simulink model "buck_ADRC_MBD_NPU_24b"  (R2025b)
settings: Solver=FixedStepAuto  StartTime=0.0  StopTime=Inf  RelTol=1e-3  EnableMultiTasking=on
InitFcn:
  | run(fullfile(fileparts(get_param(bdroot,'FileName')),'buck_npu_load_workspace.m'));
model workspace (MAT data in the model file):
  II = 0.000447333333333
  IP = 0.02847
undefined symbols (not defined in the file or in its folder): bit, Down, GPTRIP1SEL, TZ1, Up
libraries: c2802xlib x10, slpidlib x4, c28P55xlib x3, c2000lib x1
Description:
  | H15 full-convolution NPU integration: continuous 30 kHz history; background normalization/launch/result scheduling; matched-target-only LADRC correction. Boot: alpha=0, enable=1, NPU run disabled.
settings Model: ExtModeTrigDuration=8  Creator=User  LastModifiedBy=34109
settings OptimizationCC: DefaultParameterBehavior=Inlined  DefaultUnderspecifiedDataType=single  EnhancedBackFolding=on  PassReuseOutputArgsAs=Individual arguments  MaxStackSize=1024  OptimizeBlockOrder=speed  DifferentSizesBufferReuse=on  OptimizationCustomize=off  EfficientTunableParamExpr=on
settings DebuggingCC: ParameterTunabilityLossMsg=error
settings HardwareCC: ProdBitPerChar=16.0  ProdBitPerInt=16.0  ProdBitPerPointer=32.0  ProdBitPerSizeT=32.0  ProdBitPerPtrDiffT=32.0  ProdLargestAtomicInteger=Integer  ProdLargestAtomicFloat=None  ProdWordSize=16.0  ProdLongLongMode=on  ProdHWDeviceType=Texas Instruments->C2000  HardwareBoardFeatureSet=SoCBlockset
settings SFSimCC: MATLABDynamicMemAlloc=off
settings RTWCC: SystemTargetFile=ert.tlc  HardwareBoard=TI F28P55x  TemplateMakefile=ert_default_tmf  PostCodeGenCommand=buck_npu_post_codegen(buildInfo); codertarget.postCodeGenHookCommand(h);  CustomInitializer=buck_npu_platform_init();  Toolchain=Texas Instruments Code Composer Studio - EABI (C2000)  CodeProfilingSaveOptions=MetricsOnly  Description=Embedded Coder
settings RTWCC: CustomHeaderCode=|
  | #include "buck_npu.h"
  | #include "buck_npu_platform.h"
settings RTWCC: CustomInclude=|
  | C:\Users\34109\Desktop\delivery_file\F28P55_v16
  | D:/ti/c2000/C2000Ware_26_02_00_00/device_support/f28p55x/common/include
  | D:/ti/c2000/C2000Ware_26_02_00_00/driverlib/f28p55x/driverlib
settings RTWCC: CustomSource=|
  | C:\Users\34109\Desktop\delivery_file\F28P55_v16\buck_npu.c
  | C:\Users\34109\Desktop\delivery_file\F28P55_v16\buck_npu_sdk_port.c
  | C:\Users\34109\Desktop\delivery_file\F28P55_v16\buck_npu_platform.c
  | C:\Users\34109\Desktop\delivery_file\F28P55_v16\buck_load_observer.c
  | C:\Users\34109\Desktop\delivery_file\F28P55_v16\buck_npu_compensation.c
settings RTWCC: CustomLibrary=|
  | C:\Users\34109\Desktop\delivery_file\F28P55_v16\mod.a
  | C:\Users\34109\Desktop\delivery_file\F28P55_v16\buck_npu_sections.cmd
settings CodeAppCC: ForceParamTrailComments=on  IgnoreCustomStorageClasses=off  OperatorAnnotations=on  SimulinkDataObjDesc=on  SFDataObjDesc=on  InsertBlockDesc=on
settings ERTTargetCC: ExtModeTransport=4.0  ExtModeStaticAlloc=on  ExtModeAutomaticAllocSize=off  ExtModeStaticAllocSize=10000.0  ExtModeMexFile=ext_xcp  ExtModeIntrfLevel=Level2 - Open  EnableUserReplacementTypes=on  CodeReplacementLibrary=TI C28x

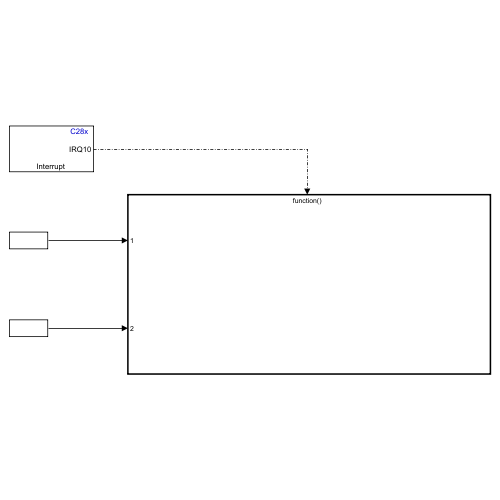
[thumbnail: Simulink's stored preview of the top-level diagram]
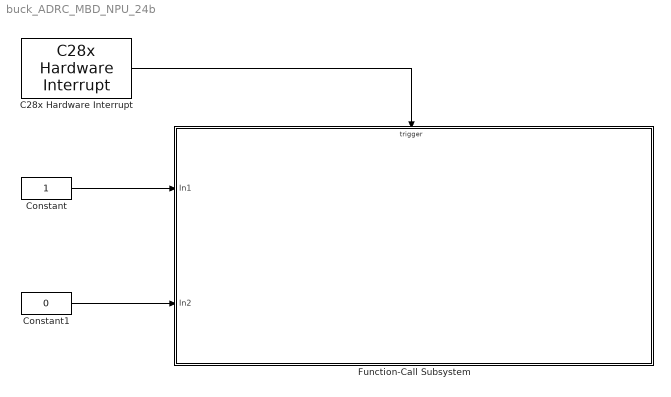
== system buck_ADRC_MBD_NPU_24b ==
  C28x Hardware Interrupt : c2000lib/Scheduling/C28x Hardware Interrupt  irqnumbers=[10]  pienumbers=[4]  irqpriorities=[30]  irqpreempts=[0]  showinput=off  dspchiptype=C280X
  Constant : Constant
  Constant1 : Constant  Value=0
  Function-Call Subsystem : Subsystem  TreatAsAtomicUnit=on
  wires:
  C28x Hardware Interrupt/1 -> Function-Call Subsystem/Trigger
  Constant1/1 -> Function-Call Subsystem/2(In2)
  Constant/1 -> Function-Call Subsystem/1(In1)

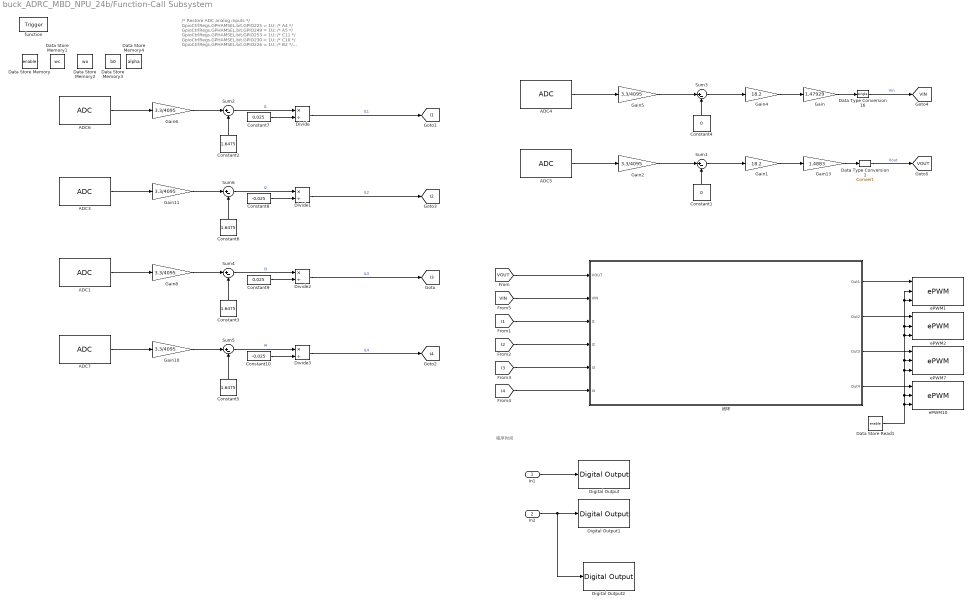
== system buck_ADRC_MBD_NPU_24b/Function-Call Subsystem ==
  note: /* Restore ADC analog inputs */
      |   GpioCtrlRegs.GPHAMSEL.bit.GPIO225 = 1U;  /* A4  */
      |   GpioCtrlRegs.GPHAMSEL.bit.GPIO249 = 1U;  /* A5  */
      |   GpioCtrlRegs.GPHAMSEL.bit.GPIO253 = 1U;  /* C11 */
      |   GpioCtrlRegs.GPHAMSEL.bit.GPIO230 = 1U;  /* C10 */
      |   GpioCtrlRegs.GPHAMSEL.bit.GPIO226 = 1U;  /* B2  */
      |   GpioCtrlRegs.GPHAMSEL.bit.GPIO237 = 1U;  /* B10 */
  note: 程序时间
  In1 : Inport
  In2 : Inport  Port=2
  function : TriggerPort  TriggerType=function-call  VariantControl=(inherit)
  ADC1 : c2802xlib/ADC  blkParamProc=C2000_Type6  ADCModule=A  samplingMode=Single sample mode  ADCResolution=12-bit (Single-ended input)  ADC29xResolution=12-bit  ADCMode=Single-ended input  useSOC1=SOC0  useSOC2=SOC0_SOC1  SOCAcquisitionWindow=56  SOCTriggerSource=ePWM7_ADCSOCA  SOCInterruptTrigger=No ADCINT  Ts=-1  dType=single  postInterrupt=off  interruptSel=ADCINT1  ADCINTContinuous=off  endma=off  chdma=1  conv1=ADCINA0  conv2=ADCINA0 and ADCINB0  conv1_Type4=ADCIN5  conv2_Type4=ADCIN0 and ADCIN1
      settings: LibrarySourceBlock=c28P55xlib/ADC
  ADC3 : c2802xlib/ADC  blkParamProc=C2000_Type6  ADCModule=C  samplingMode=Single sample mode  ADCResolution=12-bit (Single-ended input)  ADC29xResolution=12-bit  ADCMode=Single-ended input  useSOC1=SOC1  useSOC2=SOC0_SOC1  SOCAcquisitionWindow=56  SOCTriggerSource=ePWM2_ADCSOCA  SOCInterruptTrigger=No ADCINT  Ts=-1  dType=single  postInterrupt=off  interruptSel=ADCINT1  ADCINTContinuous=off  endma=off  chdma=1  conv1=ADCINA0  conv2=ADCINA0 and ADCINB0  conv1_Type4=ADCIN10  conv2_Type4=ADCIN0 and ADCIN1
      settings: LibrarySourceBlock=c28P55xlib/ADC
  ADC4 : c2802xlib/ADC  blkParamProc=C2000_Type6  ADCModule=B  samplingMode=Single sample mode  ADCResolution=12-bit (Single-ended input)  ADC29xResolution=12-bit  ADCMode=Single-ended input  useSOC1=SOC0  useSOC2=SOC0_SOC1  SOCAcquisitionWindow=56  SOCTriggerSource=ePWM1_ADCSOCA  SOCInterruptTrigger=No ADCINT  Ts=-1  dType=single  postInterrupt=off  interruptSel=ADCINT1  ADCINTContinuous=off  endma=off  chdma=1  conv1=ADCINA0  conv2=ADCINA0 and ADCINB0  conv1_Type4=ADCIN2  conv2_Type4=ADCIN0 and ADCIN1
      settings: LibrarySourceBlock=c28P55xlib/ADC
  ADC5 : c2802xlib/ADC  blkParamProc=C2000_Type6  ADCModule=B  samplingMode=Single sample mode  ADCResolution=12-bit (Single-ended input)  ADC29xResolution=12-bit  ADCMode=Single-ended input  useSOC1=SOC1  useSOC2=SOC0_SOC1  SOCAcquisitionWindow=56  SOCTriggerSource=ePWM1_ADCSOCA  SOCInterruptTrigger=No ADCINT  Ts=-1  dType=single  postInterrupt=off  interruptSel=ADCINT1  ADCINTContinuous=on  endma=off  chdma=1  conv1=ADCINA0  conv2=ADCINA0 and ADCINB0  conv1_Type4=ADCIN10  conv2_Type4=ADCIN0 and ADCIN1
      settings: LibrarySourceBlock=c28P55xlib/ADC
  ADC6 : c2802xlib/ADC  blkParamProc=C2000_Type6  ADCModule=C  samplingMode=Single sample mode  ADCResolution=12-bit (Single-ended input)  ADC29xResolution=12-bit  ADCMode=Single-ended input  useSOC1=SOC0  useSOC2=SOC0_SOC1  SOCAcquisitionWindow=56  SOCTriggerSource=ePWM1_ADCSOCA  SOCInterruptTrigger=No ADCINT  Ts=-1  dType=single  postInterrupt=off  interruptSel=ADCINT1  ADCINTContinuous=off  endma=off  chdma=1  conv1=ADCINA0  conv2=ADCINA0 and ADCINB0  conv1_Type4=ADCIN11  conv2_Type4=ADCIN0 and ADCIN1
      settings: LibrarySourceBlock=c28P55xlib/ADC
  ADC7 : c2802xlib/ADC  blkParamProc=C2000_Type6  ADCModule=A  samplingMode=Single sample mode  ADCResolution=12-bit (Single-ended input)  ADC29xResolution=12-bit  ADCMode=Single-ended input  useSOC1=SOC1  useSOC2=SOC0_SOC1  SOCAcquisitionWindow=56  SOCTriggerSource=ePWM10_ADCSOCA  SOCInterruptTrigger=No ADCINT  Ts=-1  dType=single  postInterrupt=on  interruptSel=ADCINT4  ADCINTContinuous=on  endma=off  chdma=1  conv1=ADCINA0  conv2=ADCINA0 and ADCINB0  conv1_Type4=ADCIN4  conv2_Type4=ADCIN0 and ADCIN1
      settings: LibrarySourceBlock=c28P55xlib/ADC
  Constant1 : Constant  Value=0  OutDataTypeStr=single
  Constant10 : Constant  Value=-0.025
  Constant{2..3,5..6} (4 alike) : Constant  Value=1.6475  OutDataTypeStr=single
  Constant4 : Constant  Value=0  OutDataTypeStr=single
  Constant7 : Constant  Value=0.025
  Constant8 : Constant  Value=-0.025
  Constant9 : Constant  Value=0.025
  Data Store Memory : DataStoreMemory  DataStoreName=enable  WriteAfterWriteMsg=warning  InitialValue=1  ShowAdditionalParam=off  StateMustResolveToSignalObject=on
  Data Store Memory1 : DataStoreMemory  DataStoreName=wc  WriteAfterWriteMsg=warning  InitialValue=5000  ShowAdditionalParam=off  StateMustResolveToSignalObject=on
  Data Store Memory2 : DataStoreMemory  DataStoreName=wo  WriteAfterWriteMsg=warning  InitialValue=14000  ShowAdditionalParam=off  StateMustResolveToSignalObject=on
  Data Store Memory3 : DataStoreMemory  DataStoreName=b0  WriteAfterWriteMsg=warning  InitialValue=20000  ShowAdditionalParam=off  StateMustResolveToSignalObject=on
  Data Store Memory4 : DataStoreMemory  DataStoreName=alpha  WriteAfterWriteMsg=warning  ShowAdditionalParam=off  StateMustResolveToSignalObject=on
  Data Store Read1 : DataStoreRead  DataStoreName=enable  IndexOptions=Index vector (dialog)  Indices=1  OutputSizes=1
  Data Type Conversion1 : DataTypeConversion  SaturateOnIntegerOverflow=off  RndMeth=Floor
  Data Type Conversion16 : DataTypeConversion  OutDataTypeStr=single  SaturateOnIntegerOverflow=off  RndMeth=Floor
  Digital Output : c28P55xlib/Digital Output  ExecutionOrder=First  GPIO_Number=GPIO16~GPIO23  GPIO_Bit0=off  GPIO_BIT0_Toggle=off  GPIO_Bit1=off  GPIO_BIT1_Toggle=off  GPIO_Bit2=off  GPIO_BIT2_Toggle=off  GPIO_Bit3=off  GPIO_BIT3_Toggle=off  GPIO_Bit4=off  GPIO_BIT4_Toggle=off  GPIO_Bit5=off  GPIO_BIT5_Toggle=off  GPIO_Bit6=on  GPIO_BIT6_Toggle=off  GPIO_Bit7=off  GPIO_BIT7_Toggle=off
  Digital Output1 : c28P55xlib/Digital Output  ExecutionOrder=Last  GPIO_Number=GPIO16~GPIO23  GPIO_Bit0=off  GPIO_BIT0_Toggle=off  GPIO_Bit1=off  GPIO_BIT1_Toggle=off  GPIO_Bit2=off  GPIO_BIT2_Toggle=off  GPIO_Bit3=off  GPIO_BIT3_Toggle=off  GPIO_Bit4=off  GPIO_BIT4_Toggle=off  GPIO_Bit5=off  GPIO_BIT5_Toggle=off  GPIO_Bit6=on  GPIO_BIT6_Toggle=off  GPIO_Bit7=off  GPIO_BIT7_Toggle=off
  Digital Output2 : c28P55xlib/Digital Output  GPIO_Number=GPIO56~GPIO63  GPIO_Bit0=off  GPIO_BIT0_Toggle=off  GPIO_Bit1=off  GPIO_BIT1_Toggle=off  GPIO_Bit2=off  GPIO_BIT2_Toggle=off  GPIO_Bit3=off  GPIO_BIT3_Toggle=off  GPIO_Bit4=off  GPIO_BIT4_Toggle=off  GPIO_Bit5=off  GPIO_BIT5_Toggle=off  GPIO_Bit6=off  GPIO_BIT6_Toggle=off  GPIO_Bit7=on  GPIO_BIT7_Toggle=off
  Divide{,1..3} (4 alike) : Product  Inputs=*/
  Gain : Gain  Gain=1.47929
  Gain1 : Gain  Gain=18.2
  Gain{2,5..6,8,10..11} (6 alike) : Gain  Gain=3.3/4095
  Gain13 : Gain  Gain=1.4883
  Gain4 : Gain  Gain=18.2
  Sum{1..6} (6 alike) : Sum  Inputs=|+-
  ePWM1 : c2802xlib/ePWM  PwmType=C2000_Type4_F28002x  useModule=ePWM1  ePWMxLINKTBPRD=Not Linked  periodUnits=Clock cycles  timerSource=Specify via dialog  timerPeriod_clk=2500  timerPeriod_sec=0.0001  tbshadow=Counter equals to zero  countingMode=Up-Down  phaseActiveEnable=Disable  phaseDirection=Count down after sync  phaseActive=0  synchronizationEnable=off  dcaevt1Sync=off  dcbevt1Sync=off  synchronizationOption=Disable  dcbevt1SyncOut=off  dcaevt1SyncOut=off  cmpdSyncOut=off  cmpcSyncOut=off  cmpbSyncOut=off  zeroSyncOut=on  swfSyncOut=off  perSynchronizationOption=Counter equals to period (CTR=PRD)  clockPrescale=1  HSclockPrescale=1  enswap=off  ePWMxAStatus=on  ePWMxAactionLogic1=Set  ePWMxAactionLogic2=Do nothing  ePWMxAactionLogic3=Clear  ePWMxAactionLogic4=Set  ePWMxAactionLogic5=Do nothing  ePWMxAactionLogic6=Do nothing  ePWMxACSFenable=on  ePWMxACSFvalue=Forcing disable  ePWMxASFreload=Zero  ePWMxBStatus=off  ePWMxBactionLogic1=Set  ePWMxBactionLogic2=Clear  ePWMxBactionLogic3=Do nothing  ePWMxBactionLogic4=Do nothing  ePWMxBactionLogic5=Clear  ePWMxBactionLogic6=Set  ePWMxBCSFenable=on  ePWMxBCSFvalue=Forcing disable  ePWMxBSFreload=Zero  ePWNxBOutWay=off  ePWMxLINKCMPA=Not Linked  CMPAUnits=Percentages  CMPASource=Input port  CMPAValue_per=50  CMPAValue_clk=2500  enCMPAshadow=Counter equals to zero (CTR=Zero)  ePWMxLINKCMPB=Not Linked  CMPBUnits=Clock cycles  CMPBSource=Specify via dialog  CMPBValue_per=50  CMPBValue_clk=32000  enCMPBshadow=Counter equals to zero (CTR=Zero)  ePWMxLINKCMPC=Not Linked  CMPCUnits=Clock cycles  CMPCSource=Specify via dialog  CMPCValue_per=50  CMPCValue_clk=32000  enCMPCshadow=Counter equals to zero (CTR=Zero)  ePWMxLINKCMPD=Not Linked  CMPDUnits=Clock cycles  CMPDSource=Specify via dialog  CMPDValue_per=50  CMPDValue_clk=32000  enCMPDshadow=Counter equals to zero (CTR=Zero)  enableDBePWMxA=on  enableDBePWMxB=on  enhalfcycle=off  DBpolarity=Active high complementary (AHC)  DBedgeDelay=Positive  DBSource_ePWMxA=ePWMxA  DBSource_ePWMxB=ePWMxA  DBPeriodUnits=Clock cycles  DBperiodSource=Specify via dialog  REDperiod=50  FEDperiod=50  REDperiod_sec=0  FEDperiod_sec=0  LoadModeDBRED=Immediate without using shadow  LoadModeDBFED=Immediate without using shadow  adcstartModuleA=on  adcrequestEventA=First event  adcstartEventA=Digital Compare Module A Event 1 start of conversion (DCAEVT1.soc)  adcstartEventA_type2=Counter equals to period (CTR=PRD)  adcstartModuleB=off  adcrequestEventB=First event  adcstartEventB=Counter equals to zero (CTR=Zero)  adcstartEventB_type2=Counter equals to zero (CTR=Zero)  intEn=off  intPrd=First event  intSel=Counter equals to zero (CTR=Zero)  intSel_type2=Counter equals to zero (CTR=Zero)  hrpe=off  enHRPWM=off  HRPWM_LoadMode=Counter equals to period (CTR=PRD)  HRPWM_CTLMode=Duty or Period control mode  HRPWM_EDGMode=Both edge  hrpeb=off  enHRPWMB=off  HRPWM_LoadModeB=Counter equals to zero (CTR=ZERO)  HRPWM_CTLModeB=Duty or Period control mode  HRPWM_EDGModeB=Both edge  enHRDBRED=off  enHRDBFED=off  enSFO=on  enautoconv=on  chopperEnable=off  chopperFrequency=1  chopperFirstwidth=1  chopperDuty=12.5%  tripZonesource=Specify via dialog  tzselOSHT1=off  tzselOSHT2=off  tzselOSHT3=off  tzselOSHT4=off  tzselOSHT5=off  tzselOSHT6=off  tzselOSHDCAEV1=off  tzselOSHDCBEV1=off  tzselCBC1=off  tzselCBC2=off  tzselCBC3=off  tzselCBC4=off  tzselCBC5=off  tzselCBC6=off  tzselCBCDCAEV2=off  tzselCBCDCBEV2=off  enTzOstIntr=off  enTzCbcIntr=off  enTzDCAEVT1Intr=off  enTzDCAEVT2Intr=off  enTzDCBEVT1Intr=off  enTzDCBEVT2Intr=off  tzclrCBCLatch=Counter equals to zero (CTR=Zero)  ePWMxAforced=No action  ePWMxBforced=No action  DCAEVT1forced=No action  DCBEVT1forced=No action  DCAEVT2forced=No action  DCBEVT2forced=No action  dcah=Trip Zone 1 input (TZ1)  dcal=Trip Zone 2 input (TZ2)  dcbh=Trip Zone 1 input (TZ1)  dcbl=Trip Zone 2 input (TZ2)  dcah_type2=GPTRIP1SEL/(TZ1)  dcal_type2=GPTRIP1SEL/(TZ1)  dcbh_type2=GPTRIP1SEL/(TZ1)  dcbl_type2=GPTRIP1SEL/(TZ1)  gendcaevt1=Event disabled  gendcaevt2=Event disabled  gendcbevt1=Event disabled  gendcbevt2=Event disabled  dcaevt1src=DCAEVT1 with sync  dcaevt2src=DCAEVT2 with sync  dcbevt1src=DCBEVT1 with sync  dcbevt2src=DCBEVT2 with sync  pulsesel=Counter equals to zero (CTR=Zero)  blankinv=off  blankoffset=0  blankwidth=0  evsrcsel=Filtered version of DCAEVT1 (DCAEVT1FILT)  encape=off
      settings: LibrarySourceBlock=c28P55xlib/ePWM
  ePWM10 : c2802xlib/ePWM  PwmType=C2000_Type4_F28002x  useModule=ePWM10  ePWMxLINKTBPRD=ePWM1  periodUnits=Clock cycles  timerSource=Specify via dialog  timerPeriod_clk=2500  timerPeriod_sec=0.0001  tbshadow=Counter equals to zero  countingMode=Up-Down  phaseActiveEnable=Set counter to phase value specified via dialog  phaseDirection=Count up after sync  phaseActive=1250  synchronizationEnable=off  dcaevt1Sync=off  dcbevt1Sync=off  synchronizationOption=Disable  dcbevt1SyncOut=off  dcaevt1SyncOut=off  cmpdSyncOut=off  cmpcSyncOut=off  cmpbSyncOut=off  zeroSyncOut=off  swfSyncOut=off  perSynchronizationOption=Counter equals to period (CTR=PRD)  clockPrescale=1  HSclockPrescale=1  enswap=off  ePWMxAStatus=on  ePWMxAactionLogic1=Set  ePWMxAactionLogic2=Do nothing  ePWMxAactionLogic3=Clear  ePWMxAactionLogic4=Set  ePWMxAactionLogic5=Do nothing  ePWMxAactionLogic6=Do nothing  ePWMxACSFenable=on  ePWMxACSFvalue=Forcing disable  ePWMxASFreload=Zero  ePWMxBStatus=off  ePWMxBactionLogic1=Set  ePWMxBactionLogic2=Clear  ePWMxBactionLogic3=Do nothing  ePWMxBactionLogic4=Do nothing  ePWMxBactionLogic5=Clear  ePWMxBactionLogic6=Set  ePWMxBCSFenable=on  ePWMxBCSFvalue=Forcing disable  ePWMxBSFreload=Zero  ePWNxBOutWay=off  ePWMxLINKCMPA=Not Linked  CMPAUnits=Percentages  CMPASource=Input port  CMPAValue_per=50  CMPAValue_clk=2500  enCMPAshadow=Counter equals to zero (CTR=Zero)  ePWMxLINKCMPB=Not Linked  CMPBUnits=Clock cycles  CMPBSource=Specify via dialog  CMPBValue_per=50  CMPBValue_clk=32000  enCMPBshadow=Counter equals to zero (CTR=Zero)  ePWMxLINKCMPC=Not Linked  CMPCUnits=Clock cycles  CMPCSource=Specify via dialog  CMPCValue_per=50  CMPCValue_clk=32000  enCMPCshadow=Counter equals to zero (CTR=Zero)  ePWMxLINKCMPD=Not Linked  CMPDUnits=Clock cycles  CMPDSource=Specify via dialog  CMPDValue_per=50  CMPDValue_clk=32000  enCMPDshadow=Counter equals to zero (CTR=Zero)  enableDBePWMxA=on  enableDBePWMxB=on  enhalfcycle=off  DBpolarity=Active high complementary (AHC)  DBedgeDelay=Positive  DBSource_ePWMxA=ePWMxA  DBSource_ePWMxB=ePWMxA  DBPeriodUnits=Clock cycles  DBperiodSource=Specify via dialog  REDperiod=50  FEDperiod=50  REDperiod_sec=0  FEDperiod_sec=0  LoadModeDBRED=Immediate without using shadow  LoadModeDBFED=Immediate without using shadow  adcstartModuleA=on  adcrequestEventA=First event  adcstartEventA=Digital Compare Module A Event 1 start of conversion (DCAEVT1.soc)  adcstartEventA_type2=Counter equals to period (CTR=PRD)  adcstartModuleB=off  adcrequestEventB=First event  adcstartEventB=Counter equals to zero (CTR=Zero)  adcstartEventB_type2=Counter equals to zero (CTR=Zero)  intEn=off  intPrd=First event  intSel=Counter equals to zero (CTR=Zero)  intSel_type2=Counter equals to zero (CTR=Zero)  hrpe=off  enHRPWM=off  HRPWM_LoadMode=Counter equals to period (CTR=PRD)  HRPWM_CTLMode=Duty or Period control mode  HRPWM_EDGMode=Both edge  hrpeb=off  enHRPWMB=off  HRPWM_LoadModeB=Counter equals to zero (CTR=ZERO)  HRPWM_CTLModeB=Duty or Period control mode  HRPWM_EDGModeB=Both edge  enHRDBRED=off  enHRDBFED=off  enSFO=on  enautoconv=on  chopperEnable=off  chopperFrequency=1  chopperFirstwidth=1  chopperDuty=12.5%  tripZonesource=Specify via dialog  tzselOSHT1=off  tzselOSHT2=off  tzselOSHT3=off  tzselOSHT4=off  tzselOSHT5=off  tzselOSHT6=off  tzselOSHDCAEV1=off  tzselOSHDCBEV1=off  tzselCBC1=off  tzselCBC2=off  tzselCBC3=off  tzselCBC4=off  tzselCBC5=off  tzselCBC6=off  tzselCBCDCAEV2=off  tzselCBCDCBEV2=off  enTzOstIntr=off  enTzCbcIntr=off  enTzDCAEVT1Intr=off  enTzDCAEVT2Intr=off  enTzDCBEVT1Intr=off  enTzDCBEVT2Intr=off  tzclrCBCLatch=Counter equals to zero (CTR=Zero)  ePWMxAforced=No action  ePWMxBforced=No action  DCAEVT1forced=No action  DCBEVT1forced=No action  DCAEVT2forced=No action  DCBEVT2forced=No action  dcah=Trip Zone 1 input (TZ1)  dcal=Trip Zone 2 input (TZ2)  dcbh=Trip Zone 1 input (TZ1)  dcbl=Trip Zone 2 input (TZ2)  dcah_type2=GPTRIP1SEL/(TZ1)  dcal_type2=GPTRIP1SEL/(TZ1)  dcbh_type2=GPTRIP1SEL/(TZ1)  dcbl_type2=GPTRIP1SEL/(TZ1)  gendcaevt1=Event disabled  gendcaevt2=Event disabled  gendcbevt1=Event disabled  gendcbevt2=Event disabled  dcaevt1src=DCAEVT1 with sync  dcaevt2src=DCAEVT2 with sync  dcbevt1src=DCBEVT1 with sync  dcbevt2src=DCBEVT2 with sync  pulsesel=Counter equals to zero (CTR=Zero)  blankinv=off  blankoffset=0  blankwidth=0  evsrcsel=Filtered version of DCAEVT1 (DCAEVT1FILT)  encape=off
      settings: LibrarySourceBlock=c28P55xlib/ePWM
  ePWM2 : c2802xlib/ePWM  PwmType=C2000_Type4_F28002x  useModule=ePWM2  ePWMxLINKTBPRD=Not Linked  periodUnits=Clock cycles  timerSource=Specify via dialog  timerPeriod_clk=2500  timerPeriod_sec=0.0001  tbshadow=Counter equals to zero  countingMode=Up-Down  phaseActiveEnable=Set counter to phase value specified via dialog  phaseDirection=Count down after sync  phaseActive=1250  synchronizationEnable=off  dcaevt1Sync=off  dcbevt1Sync=off  synchronizationOption=Disable  dcbevt1SyncOut=off  dcaevt1SyncOut=off  cmpdSyncOut=off  cmpcSyncOut=off  cmpbSyncOut=off  zeroSyncOut=off  swfSyncOut=off  perSynchronizationOption=Counter equals to period (CTR=PRD)  clockPrescale=1  HSclockPrescale=1  enswap=off  ePWMxAStatus=on  ePWMxAactionLogic1=Set  ePWMxAactionLogic2=Do nothing  ePWMxAactionLogic3=Clear  ePWMxAactionLogic4=Set  ePWMxAactionLogic5=Do nothing  ePWMxAactionLogic6=Do nothing  ePWMxACSFenable=on  ePWMxACSFvalue=Forcing disable  ePWMxASFreload=Zero  ePWMxBStatus=off  ePWMxBactionLogic1=Set  ePWMxBactionLogic2=Clear  ePWMxBactionLogic3=Do nothing  ePWMxBactionLogic4=Do nothing  ePWMxBactionLogic5=Clear  ePWMxBactionLogic6=Set  ePWMxBCSFenable=on  ePWMxBCSFvalue=Forcing disable  ePWMxBSFreload=Zero  ePWNxBOutWay=off  ePWMxLINKCMPA=Not Linked  CMPAUnits=Percentages  CMPASource=Input port  CMPAValue_per=50  CMPAValue_clk=2500  enCMPAshadow=Counter equals to zero (CTR=Zero)  ePWMxLINKCMPB=Not Linked  CMPBUnits=Clock cycles  CMPBSource=Specify via dialog  CMPBValue_per=50  CMPBValue_clk=32000  enCMPBshadow=Counter equals to zero (CTR=Zero)  ePWMxLINKCMPC=Not Linked  CMPCUnits=Clock cycles  CMPCSource=Specify via dialog  CMPCValue_per=50  CMPCValue_clk=32000  enCMPCshadow=Counter equals to zero (CTR=Zero)  ePWMxLINKCMPD=Not Linked  CMPDUnits=Clock cycles  CMPDSource=Specify via dialog  CMPDValue_per=50  CMPDValue_clk=32000  enCMPDshadow=Counter equals to zero (CTR=Zero)  enableDBePWMxA=on  enableDBePWMxB=on  enhalfcycle=off  DBpolarity=Active high complementary (AHC)  DBedgeDelay=Positive  DBSource_ePWMxA=ePWMxA  DBSource_ePWMxB=ePWMxA  DBPeriodUnits=Clock cycles  DBperiodSource=Specify via dialog  REDperiod=50  FEDperiod=50  REDperiod_sec=0  FEDperiod_sec=0  LoadModeDBRED=Immediate without using shadow  LoadModeDBFED=Immediate without using shadow  adcstartModuleA=on  adcrequestEventA=First event  adcstartEventA=Digital Compare Module A Event 1 start of conversion (DCAEVT1.soc)  adcstartEventA_type2=Counter equals to period (CTR=PRD)  adcstartModuleB=off  adcrequestEventB=First event  adcstartEventB=Counter equals to zero (CTR=Zero)  adcstartEventB_type2=Counter equals to zero (CTR=Zero)  intEn=off  intPrd=First event  intSel=Counter equals to zero (CTR=Zero)  intSel_type2=Counter equals to zero (CTR=Zero)  hrpe=off  enHRPWM=off  HRPWM_LoadMode=Counter equals to period (CTR=PRD)  HRPWM_CTLMode=Duty or Period control mode  HRPWM_EDGMode=Both edge  hrpeb=off  enHRPWMB=off  HRPWM_LoadModeB=Counter equals to zero (CTR=ZERO)  HRPWM_CTLModeB=Duty or Period control mode  HRPWM_EDGModeB=Both edge  enHRDBRED=off  enHRDBFED=off  enSFO=on  enautoconv=on  chopperEnable=off  chopperFrequency=1  chopperFirstwidth=1  chopperDuty=12.5%  tripZonesource=Specify via dialog  tzselOSHT1=off  tzselOSHT2=off  tzselOSHT3=off  tzselOSHT4=off  tzselOSHT5=off  tzselOSHT6=off  tzselOSHDCAEV1=off  tzselOSHDCBEV1=off  tzselCBC1=off  tzselCBC2=off  tzselCBC3=off  tzselCBC4=off  tzselCBC5=off  tzselCBC6=off  tzselCBCDCAEV2=off  tzselCBCDCBEV2=off  enTzOstIntr=off  enTzCbcIntr=off  enTzDCAEVT1Intr=off  enTzDCAEVT2Intr=off  enTzDCBEVT1Intr=off  enTzDCBEVT2Intr=off  tzclrCBCLatch=Counter equals to zero (CTR=Zero)  ePWMxAforced=No action  ePWMxBforced=No action  DCAEVT1forced=No action  DCBEVT1forced=No action  DCAEVT2forced=No action  DCBEVT2forced=No action  dcah=Trip Zone 1 input (TZ1)  dcal=Trip Zone 2 input (TZ2)  dcbh=Trip Zone 1 input (TZ1)  dcbl=Trip Zone 2 input (TZ2)  dcah_type2=GPTRIP1SEL/(TZ1)  dcal_type2=GPTRIP1SEL/(TZ1)  dcbh_type2=GPTRIP1SEL/(TZ1)  dcbl_type2=GPTRIP1SEL/(TZ1)  gendcaevt1=Event disabled  gendcaevt2=Event disabled  gendcbevt1=Event disabled  gendcbevt2=Event disabled  dcaevt1src=DCAEVT1 with sync  dcaevt2src=DCAEVT2 with sync  dcbevt1src=DCBEVT1 with sync  dcbevt2src=DCBEVT2 with sync  pulsesel=Counter equals to zero (CTR=Zero)  blankinv=off  blankoffset=0  blankwidth=0  evsrcsel=Filtered version of DCAEVT1 (DCAEVT1FILT)  encape=off
      settings: LibrarySourceBlock=c28P55xlib/ePWM
  ePWM7 : c2802xlib/ePWM  PwmType=C2000_Type4_F28002x  useModule=ePWM7  ePWMxLINKTBPRD=ePWM1  periodUnits=Clock cycles  timerSource=Specify via dialog  timerPeriod_clk=2500  timerPeriod_sec=0.0001  tbshadow=Counter equals to zero  countingMode=Up-Down  phaseActiveEnable=Set counter to phase value specified via dialog  phaseDirection=Count up after sync  phaseActive=2500  synchronizationEnable=off  dcaevt1Sync=off  dcbevt1Sync=off  synchronizationOption=Disable  dcbevt1SyncOut=off  dcaevt1SyncOut=off  cmpdSyncOut=off  cmpcSyncOut=off  cmpbSyncOut=off  zeroSyncOut=off  swfSyncOut=off  perSynchronizationOption=Counter equals to period (CTR=PRD)  clockPrescale=1  HSclockPrescale=1  enswap=off  ePWMxAStatus=on  ePWMxAactionLogic1=Set  ePWMxAactionLogic2=Do nothing  ePWMxAactionLogic3=Clear  ePWMxAactionLogic4=Set  ePWMxAactionLogic5=Do nothing  ePWMxAactionLogic6=Do nothing  ePWMxACSFenable=on  ePWMxACSFvalue=Forcing disable  ePWMxASFreload=Zero  ePWMxBStatus=off  ePWMxBactionLogic1=Set  ePWMxBactionLogic2=Clear  ePWMxBactionLogic3=Do nothing  ePWMxBactionLogic4=Do nothing  ePWMxBactionLogic5=Clear  ePWMxBactionLogic6=Set  ePWMxBCSFenable=on  ePWMxBCSFvalue=Forcing disable  ePWMxBSFreload=Zero  ePWNxBOutWay=off  ePWMxLINKCMPA=Not Linked  CMPAUnits=Percentages  CMPASource=Input port  CMPAValue_per=50  CMPAValue_clk=2500  enCMPAshadow=Counter equals to zero (CTR=Zero)  ePWMxLINKCMPB=Not Linked  CMPBUnits=Clock cycles  CMPBSource=Specify via dialog  CMPBValue_per=50  CMPBValue_clk=32000  enCMPBshadow=Counter equals to zero (CTR=Zero)  ePWMxLINKCMPC=Not Linked  CMPCUnits=Clock cycles  CMPCSource=Specify via dialog  CMPCValue_per=50  CMPCValue_clk=32000  enCMPCshadow=Counter equals to zero (CTR=Zero)  ePWMxLINKCMPD=Not Linked  CMPDUnits=Clock cycles  CMPDSource=Specify via dialog  CMPDValue_per=50  CMPDValue_clk=32000  enCMPDshadow=Counter equals to zero (CTR=Zero)  enableDBePWMxA=on  enableDBePWMxB=on  enhalfcycle=off  DBpolarity=Active high complementary (AHC)  DBedgeDelay=Positive  DBSource_ePWMxA=ePWMxA  DBSource_ePWMxB=ePWMxA  DBPeriodUnits=Clock cycles  DBperiodSource=Specify via dialog  REDperiod=50  FEDperiod=50  REDperiod_sec=0  FEDperiod_sec=0  LoadModeDBRED=Immediate without using shadow  LoadModeDBFED=Immediate without using shadow  adcstartModuleA=on  adcrequestEventA=First event  adcstartEventA=Digital Compare Module A Event 1 start of conversion (DCAEVT1.soc)  adcstartEventA_type2=Counter equals to period (CTR=PRD)  adcstartModuleB=off  adcrequestEventB=First event  adcstartEventB=Counter equals to zero (CTR=Zero)  adcstartEventB_type2=Counter equals to zero (CTR=Zero)  intEn=off  intPrd=First event  intSel=Counter equals to zero (CTR=Zero)  intSel_type2=Counter equals to zero (CTR=Zero)  hrpe=off  enHRPWM=off  HRPWM_LoadMode=Counter equals to period (CTR=PRD)  HRPWM_CTLMode=Duty or Period control mode  HRPWM_EDGMode=Both edge  hrpeb=off  enHRPWMB=off  HRPWM_LoadModeB=Counter equals to zero (CTR=ZERO)  HRPWM_CTLModeB=Duty or Period control mode  HRPWM_EDGModeB=Both edge  enHRDBRED=off  enHRDBFED=off  enSFO=on  enautoconv=on  chopperEnable=off  chopperFrequency=1  chopperFirstwidth=1  chopperDuty=12.5%  tripZonesource=Specify via dialog  tzselOSHT1=off  tzselOSHT2=off  tzselOSHT3=off  tzselOSHT4=off  tzselOSHT5=off  tzselOSHT6=off  tzselOSHDCAEV1=off  tzselOSHDCBEV1=off  tzselCBC1=off  tzselCBC2=off  tzselCBC3=off  tzselCBC4=off  tzselCBC5=off  tzselCBC6=off  tzselCBCDCAEV2=off  tzselCBCDCBEV2=off  enTzOstIntr=off  enTzCbcIntr=off  enTzDCAEVT1Intr=off  enTzDCAEVT2Intr=off  enTzDCBEVT1Intr=off  enTzDCBEVT2Intr=off  tzclrCBCLatch=Counter equals to zero (CTR=Zero)  ePWMxAforced=No action  ePWMxBforced=No action  DCAEVT1forced=No action  DCBEVT1forced=No action  DCAEVT2forced=No action  DCBEVT2forced=No action  dcah=Trip Zone 1 input (TZ1)  dcal=Trip Zone 2 input (TZ2)  dcbh=Trip Zone 1 input (TZ1)  dcbl=Trip Zone 2 input (TZ2)  dcah_type2=GPTRIP1SEL/(TZ1)  dcal_type2=GPTRIP1SEL/(TZ1)  dcbh_type2=GPTRIP1SEL/(TZ1)  dcbl_type2=GPTRIP1SEL/(TZ1)  gendcaevt1=Event disabled  gendcaevt2=Event disabled  gendcbevt1=Event disabled  gendcbevt2=Event disabled  dcaevt1src=DCAEVT1 with sync  dcaevt2src=DCAEVT2 with sync  dcbevt1src=DCBEVT1 with sync  dcbevt2src=DCBEVT2 with sync  pulsesel=Counter equals to zero (CTR=Zero)  blankinv=off  blankoffset=0  blankwidth=0  evsrcsel=Filtered version of DCAEVT1 (DCAEVT1FILT)  encape=off
      settings: LibrarySourceBlock=c28P55xlib/ePWM
  闭环 : Subsystem
  tag scope: I1=global, I2=global, I3=global, I4=global, VIN=global, VOUT=global
  wires:
  Data Type Conversion16/1 -> [VIN]  "Vin"
  [I2] -> 闭环/4(I2)
  ADC5/1 -> Gain2/1
  Data Type Conversion1/1 -> [VOUT]  "Vout"
  Gain1/1 -> Gain13/1
  Gain5/1 -> Sum3/1
  Constant1/1 -> Sum1/2
  [VOUT] -> 闭环/1(VOUT)
  Gain2/1 -> Sum1/1
  [I3] -> 闭环/5(I3)
  [I4] -> 闭环/6(I4)
  ADC4/1 -> Gain5/1
  Sum1/1 -> Gain1/1
  Constant4/1 -> Sum3/2
  Sum3/1 -> Gain4/1
  [I1] -> 闭环/3(I1)
  Gain6/1 -> Sum2/1
  Constant2/1 -> Sum2/2
  Divide/1 -> [I1]  "IL1"
  Constant3/1 -> Sum4/2
  Gain8/1 -> Sum4/1
  Divide3/1 -> [I4]  "IL4"
  Gain10/1 -> Sum5/1
  Constant5/1 -> Sum5/2
  Constant6/1 -> Sum6/2
  Gain11/1 -> Sum6/1
  Divide1/1 -> [I2]  "IL2"
  Gain/1 -> Data Type Conversion16/1
  Gain4/1 -> Gain/1
  Gain13/1 -> Data Type Conversion1/1
  Divide2/1 -> [I3]  "IL3"
  Sum2/1 -> Divide/1  "I1"
  Constant7/1 -> Divide/2
  Sum6/1 -> Divide1/1  "I2"
  Constant8/1 -> Divide1/2
  Constant9/1 -> Divide2/2
  Sum4/1 -> Divide2/1  "I3"
  Sum5/1 -> Divide3/1  "I4"
  Constant10/1 -> Divide3/2
  闭环/3(Out3) -> ePWM7/1
  闭环/2(Out2) -> ePWM2/1
  闭环/4(Out4) -> ePWM10/1
  闭环/1(Out1) -> ePWM1/1
  Data Store Read1/1 -> ePWM2/3, ePWM2/2, ePWM1/3, ePWM1/2, ePWM7/2, ePWM7/3, ePWM10/2, ePWM10/3
  ADC6/1 -> Gain6/1
  ADC3/1 -> Gain11/1
  ADC1/1 -> Gain8/1
  ADC7/1 -> Gain10/1
  [VIN] -> 闭环/2(VIN)
  In2/1 -> Digital Output1/1, Digital Output2/1
  In1/1 -> Digital Output/1

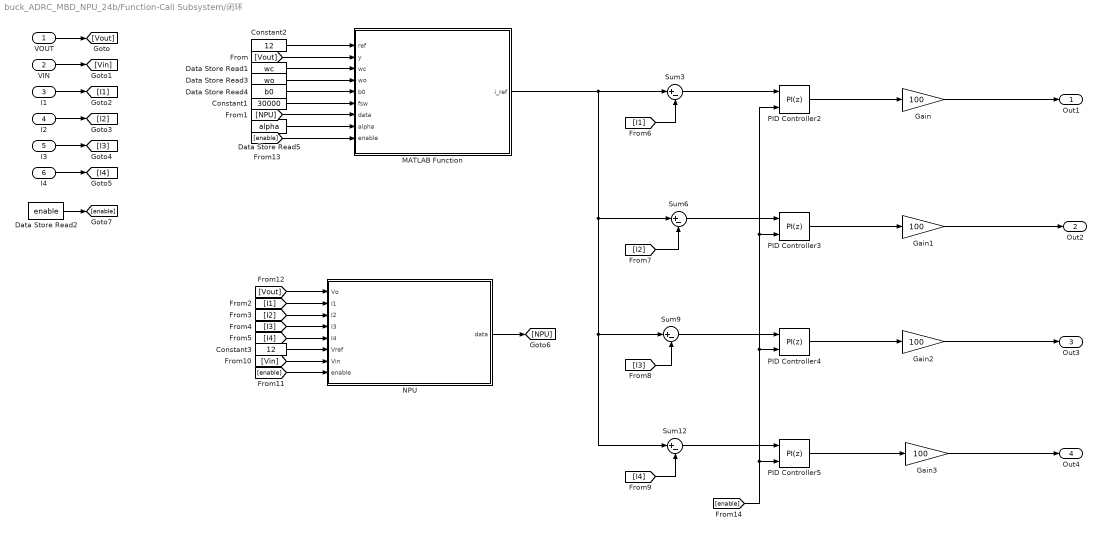
== system buck_ADRC_MBD_NPU_24b/Function-Call Subsystem/闭环 ==
  VOUT : Inport
  VIN : Inport  Port=2
  I1 : Inport  Port=3
  I2 : Inport  Port=4
  I3 : Inport  Port=5
  I4 : Inport  Port=6
  Constant1 : Constant  Value=30000
  Constant2 : Constant  Value=12
  Constant3 : Constant  Value=12
  Data Store Read1 : DataStoreRead  DataStoreName=wc  IndexOptions=Index vector (dialog)  Indices=1  OutputSizes=1
  Data Store Read2 : DataStoreRead  DataStoreName=enable  IndexOptions=Index vector (dialog)  Indices=1  OutputSizes=1
  Data Store Read3 : DataStoreRead  DataStoreName=wo  IndexOptions=Index vector (dialog)  Indices=1  OutputSizes=1
  Data Store Read4 : DataStoreRead  DataStoreName=b0  IndexOptions=Index vector (dialog)  Indices=1  OutputSizes=1
  Data Store Read5 : DataStoreRead  DataStoreName=alpha  IndexOptions=Index vector (dialog)  Indices=1  OutputSizes=1
  Gain{,1..3} (4 alike) : Gain  Gain=100
  MATLAB Function : MATLAB Function  TreatAsAtomicUnit=on
  NPU : MATLAB Function  TreatAsAtomicUnit=on
  PID Controller{2..5} (4 alike) : slpidlib/PID Controller  Controller=PI  Form=Parallel  TimeDomain=Discrete-time  UseExternalTs=off  SampleTime=-1  IntegratorMethod=Forward Euler  FilterMethod=Forward Euler  ControllerParametersSource=internal  P=0.1  I=0.00025  UseKiTs=on  D=0  UseExternalDerivativeSource=off  N=100  UseFilter=on  TunerSelectOption=Transfer Function Based (PID Tuner App)  InitialConditionSource=internal  InitialConditionForIntegrator=0.05  InitialConditionForFilter=0  DifferentiatorICPrevScaledInput=0  ExternalReset=either  TrackingMode=off  Kt=1  LimitOutput=on  SatLimitsSource=internal  UpperSaturationLimit=0.95  LowerSaturationLimit=0.05  LinearizeAsGain=on  AntiWindupMode=clamping  Kb=1  LimitIntegrator=off  UpperIntegratorSaturationLimit=inf  LowerIntegratorSaturationLimit=-inf  POutMin=[]  POutMax=[]  IOutMin=[]  IOutMax=[]  DOutMin=[]  DOutMax=[]  NOutMin=[]  NOutMax=[]  SumOutMin=[]  SumOutMax=[]  SaturationOutMin=[]  SaturationOutMax=[]  PParamMin=[]  PParamMax=[]  IParamMin=[]  IParamMax=[]  DParamMin=[]  DParamMax=[]  NParamMin=[]  NParamMax=[]  KbParamMin=[]  KbParamMax=[]  KtParamMin=[]  KtParamMax=[]  KbOutMin=[]  KbOutMax=[]  KtOutMin=[]  KtOutMax=[]  IntegratorOutMin=[]  IntegratorOutMax=[]  FilterOutMin=[]  FilterOutMax=[]  SumI1OutMin=[]  SumI1OutMax=[]  SumI2OutMin=[]  SumI2OutMax=[]  SumI3OutMin=[]  SumI3OutMax=[]  SumI4OutMin=[]  SumI4OutMax=[]  SumDOutMin=[]  SumDOutMax=[]  DifferentiatorOutMin=[]  DifferentiatorOutMax=[]  FilterDiffOutCoefMin=[]  FilterDiffOutCoefMax=[]  ReciprocalOutMin=[]  ReciprocalOutMax=[]  SumDenOutMin=[]  SumDenOutMax=[]  SumNumOutMin=[]  SumNumOutMax=[]  DivideOutMin=[]  DivideOutMax=[]  UdiffTsProdOutMin=[]  UdiffTsProdOutMax=[]  NTsProdOutMin=[]  NTsProdOutMax=[]  UintegralTsProdOutMin=[]  UintegralTsProdOutMax=[]  UngainTsProdOutMin=[]  UngainTsProdOutMax=[]  ClampingZeroOutDataTypeStr=Inherit: Inherit via back propagation  ClampingZeroOutMin=[]  ClampingZeroOutMax=[]  FilterDenConstantOutDataTypeStr=Inherit: Inherit via back propagation  FilterDenConstantOutMin=[]  FilterDenConstantOutMax=[]  PCopyOutDataTypeStr=Inherit: Inherit via back propagation  PCopyOutMin=[]  PCopyOutMax=[]  NCopyOutDataTypeStr=Inherit: Inherit via back propagation  NCopyOutMin=[]  NCopyOutMax=[]  IntegratorContinuousStateAttributes=''  IntegratorStateMustResolveToSignalObject=off  IntegratorRTWStateStorageClass=Auto  FilterContinuousStateAttributes=''  FilterStateMustResolveToSignalObject=off  FilterRTWStateStorageClass=Auto  ParallelPVariant=InternalParameters  IdealPVariant=Disabled  IVariant=InternalParameters  DVariant=Disabled  IntegratorVariant=Discrete  SatVariant=Enabled  AWVariant=DiscClampingParallel  PCopyVariant=Disabled  TRVariant=Disabled  FdbkBlocksVariant=Forward  IdealPFdbkVariant=Disabled  SatFdbkVariant=Disabled  DerivativeFilterVariant=Disabled  NVariant=Disabled  NCopyVariant=Disabled_SignalSpec  FilterICVariant=Disabled  IntegratorICVariant=InternalICs  ExternalResetVariant=ExternalReset  TRSumVariant=Passthrough  SumFdbkVariant=Disabled  SumVariant=Sum_PI  TsampFilterVariant=InternalTs  TsampNgainVariant=Passthrough  TsampIntegralVariant=Disabled_SignalSpec  ExternalSaturationOutDataTypeStr=Inherit: Same as second input  DerivativeSourceVariant=Disabled  PreIntVariant=InternalPreInt
  Sum{3,6,9,12} (4 alike) : Sum  Inputs=|+-
  Out1 : Outport
  Out2 : Outport  Port=2
  Out3 : Outport  Port=3
  Out4 : Outport  Port=4
  wires:
  PID Controller2/1 -> Gain/1
  Sum3/1 -> PID Controller2/1
  PID Controller3/1 -> Gain1/1
  Sum9/1 -> PID Controller4/1
  PID Controller4/1 -> Gain2/1
  PID Controller5/1 -> Gain3/1
  Sum6/1 -> PID Controller3/1
  Sum12/1 -> PID Controller5/1
  MATLAB Function/1(i_ref) -> Sum12/1, Sum9/1, Sum6/1, Sum3/1
  Constant1/1 -> MATLAB Function/6(fsw)
  Data Store Read4/1 -> MATLAB Function/5(b0)
  Data Store Read1/1 -> MATLAB Function/3(wc)
  Data Store Read3/1 -> MATLAB Function/4(wo)
  Constant2/1 -> MATLAB Function/1(ref)
  Gain3/1 -> Out4/1
  Gain/1 -> Out1/1
  Gain1/1 -> Out2/1
  Gain2/1 -> Out3/1
  VOUT/1 -> [Vout]
  VIN/1 -> [Vin]
  I1/1 -> [I1]
  I2/1 -> [I2]
  I3/1 -> [I3]
  I4/1 -> [I4]
  [Vout] -> MATLAB Function/2(y)
  NPU/1(data) -> [NPU]
  [NPU] -> MATLAB Function/7(data)
  [I2] -> NPU/3(I2)
  [I3] -> NPU/4(I3)
  [I4] -> NPU/5(I4)
  [I1] -> NPU/2(I1)
  [I4] -> Sum12/2
  [I3] -> Sum9/2
  [I2] -> Sum6/2
  [I1] -> Sum3/2
  [Vin] -> NPU/7(Vin)
  Constant3/1 -> NPU/6(Vref)
  Data Store Read2/1 -> [enable]
  [enable] -> NPU/8(enable)
  [Vout] -> NPU/1(Vo)
  [enable] -> MATLAB Function/9(enable)
  [enable] -> PID Controller2/2, PID Controller3/2, PID Controller4/2, PID Controller5/2
  Data Store Read5/1 -> MATLAB Function/8(alpha)

== matlab function buck_ADRC_MBD_NPU_24b/Function-Call Subsystem/闭环/NPU ==
  data: data output; Vo input; I1 input; I2 input; I3 input; I4 input; Vref input; Vin input; enable input
function data = NPU(Vo,I1,I2,I3,I4,Vref,Vin,enable)
%#codegen
% v15 CPU 采样/负载电流观测/已排定事件读取接口；不等待 NPU。
% 输出是配对端点的扰动变化量 df（V/s），交给 ADRC 内的
% buck_npu_apply_prediction 使用；不能直接与当前 z2 相减。
% enable=1 复位，0 运行。普通桌面仿真使用 NaN -> 原 ADRC。
data = single(NaN);
if coder.target('Rtw')
    coder.cinclude('buck_npu.h');
    data = coder.ceval('buck_npu_begin',single(Vo),single(I1),single(I2), ...
        single(I3),single(I4),single(Vref),single(Vin),uint16(enable~=0));
end
end

== matlab function buck_ADRC_MBD_NPU_24b/Function-Call Subsystem/闭环/MATLAB Function ==
  data: ref input; i_ref output; y input; wc input; wo input; b0 input; fsw input; data input; alpha input; enable input
function i_ref = Voltage_ADRC(ref, y, wc, wo, b0, fsw, data, alpha, enable)
%#codegen
% v15：一阶 LADRC 电压外环，输出每相电感电流给定（A）。
% 保留原来的 9 个输入、1 个输出及原 ESO/电流限幅算法。
% data 是上一负载周期配对端点的总扰动变化量 df（V/s），不是当前 z2。
% v15 C 接口完成提前前馈及 ESO 接管；不能再直接计算 (data-z2)。
% enable=1：复位；enable=0：运行。alpha=0：补偿为零。
% 本函数只读取/使用预测并提交采样，不执行或等待神经网络推理。

persistent z1 z2 u_prev
ref_s = single(ref); y_s = single(y);
wc_s = single(wc); wo_s = single(wo); b0_s = single(b0);
fsw_s = single(fsw);
zero = single(0); Imax = single(40);
alpha_s = single(alpha);
if ~isfinite(alpha_s)
    alpha_s = zero;
else
    alpha_s = min(max(alpha_s,zero),single(1));
end
if isempty(z1)
    z1 = y_s; z2 = zero; u_prev = zero;
end
reset = enable ~= 0;
if ~isfinite(fsw_s) || fsw_s <= zero || ~isfinite(b0_s) || abs(b0_s) < single(1e-6)
    reset = true;
end
if coder.target('Rtw')
    coder.cinclude('buck_npu.h');
    coder.cinclude('buck_npu_mbd_bridge.h');
end
if reset
    z1 = y_s; z2 = zero; u_prev = zero;
    cmd = zero;
    if coder.target('Rtw')
        coder.ceval('buck_npu_mbd_record_reset');
    end
else
    Ts = single(1)/fsw_s;
    % 原 ESO：使用上一周期最终限幅后的电流给定。
    e = y_s-z1;
    z1 = z1+Ts*(z2+b0_s*u_prev+single(2)*wo_s*e);
    z2 = z2+Ts*(wo_s*wo_s*e);

    % 每个运行周期都调用，使 alpha=0/失锁/停用等条件能取消旧补偿。
    % 必须在本周期 ESO 更新之后调用，保持 v15 的交还时序。
    delta_I = zero;
    if coder.target('Rtw')
        delta_I = coder.ceval('buck_npu_apply_prediction',single(data),single(z2), ...
            alpha_s,b0_s,wc_s,wo_s);
    end
    raw = (wc_s*(ref_s-z1)-z2)/b0_s;
    if coder.target('Rtw')
        coder.ceval('buck_npu_mbd_record_baseline',single(raw));
    end
    cmd = min(max(raw+delta_I,-Imax),Imax);
    if coder.target('Rtw')
        coder.ceval('buck_npu_mbd_record_final',single(cmd));
    end
    u_prev = cmd;
end
i_ref = double(cmd);
% 收集本周期真实控制量与 ESO 状态；推理仍由 main 后台服务。
if coder.target('Rtw')
    coder.ceval('buck_npu_commit',single(cmd),single(z2),fsw_s,b0_s,uint16(reset));
end
end
